simulink model "sf_boiler"  (R2025b)
settings: Solver=ode45  StartTime=0.0  StopTime=1400  RelTol=1e-3  EnableMultiTasking=on
settings Model: ExtModeTrigMode=oneshot  ExtModeArmWhenConnect=off  ExtModeAutoUpdateStatusClock=off  Creator=The MathWorks, Inc.  LastModifiedBy=The MathWorks, Inc.
settings SolverCC: AlgebraicLoopSolver=TrustRegion  InsertRTBMode=Auto
settings DataIOCC: SaveFormat=Array  SaveOutput=off  SaveTime=off  ReturnWorkspaceOutputs=off  SignalLoggingName=sigsOut
settings OptimizationCC: BlockReduction=off  BooleanDataType=off  ReuseModelBlockBuffer=off  ExpressionDepthLimit=2147483647.0  InitFltsAndDblsToZero=on  LifeSpan=1  EfficientTunableParamExpr=on
settings DebuggingCC: SaveWithParameterizedLinksMsg=none  UnderspecifiedInitializationDetection=Classic  MergeDetectMultiDrivingBlocksExec=none  SignalResolutionControl=TryResolveAllWithWarning  MultiTaskDSMMsg=warning  MultiTaskCondExecSysMsg=none  FcnCallInpInsideContextMsg=warning  UnconnectedInputMsg=warning  UnconnectedOutputMsg=warning  UnconnectedLineMsg=warning  StateNameClashWarn=warning  SFUnexpectedBacktrackingDiag=warning  SFNoUnconditionalDefaultTransitionDiag=warning  SFExecutionAtInitializationDiag=none  ArithmeticOperatorsInVariantConditions=warning
settings HardwareCC: ProdBitPerPointer=32.0  ProdBitPerSizeT=32.0  ProdBitPerPtrDiffT=32.0  ProdLargestAtomicFloat=None  ProdIntDivRoundTo=Undefined  ProdEndianess=Unspecified  ProdWordSize=32.0  ProdHWDeviceType=ASIC/FPGA  TargetUnknown=on  ProdEqTarget=off
settings ModelReferenceCC: EnableRefExpFcnMdlSchedulingChecks=on  PropagateSignalLabelsOutOfModel=off
settings SFSimCC: SFSimEcho=off  SimUseLocalCustomCode=off  SimParseCustomCode=off  CustomCodeUndefinedFunction=UseInterfaceOnly
settings RTWCC: SystemTargetFile=ert.tlc  GenCodeOnly=on  TemplateMakefile=ert_default_tmf  GenerateReport=on  RTWVerbose=off  RTWUseLocalCustomCode=off  IncludeHyperlinkInReport=on  LaunchReport=on  GPUComputeCapability=3.5  DLArmComputeVersion=19.05
settings CodeAppCC: IgnoreCustomStorageClasses=off  CustomSymbolStrType=$N$R$M  CustomSymbolStrModelFcn=$N  StateflowObjectComments=on  InternalIdentifier=Classic
settings ERTTargetCC: InlinedParameterPlacement=Hierarchical  ERTCustomFileTemplate=example_file_process.tlc  ConvertIfToSwitch=off  SuppressUnreachableDefaultCases=off  TargetFcnLib=ansi_tfl_tmw.mat  MultiwordLength=2048.0  GenerateSampleERTMain=on  SupportContinuousTime=on  SupportNonInlinedSFcns=on
settings ConfigComp: CovMetricSettings=dcmtr  CovSaveCumulativeToWorkspaceVar=on  CovSaveSingleToWorkspaceVar=on  CovExternalEMLEnable=off  CovSFcnEnable=off

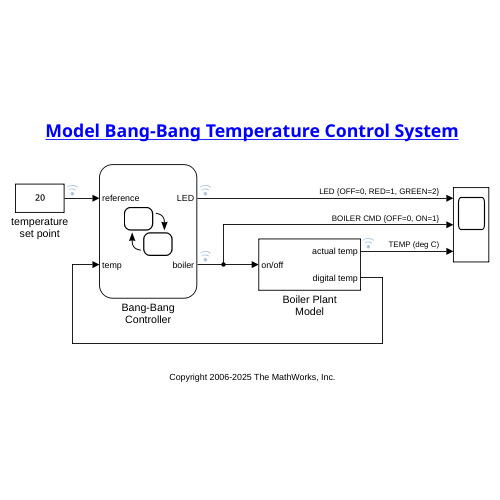
[thumbnail: Simulink's stored preview of the top-level diagram]
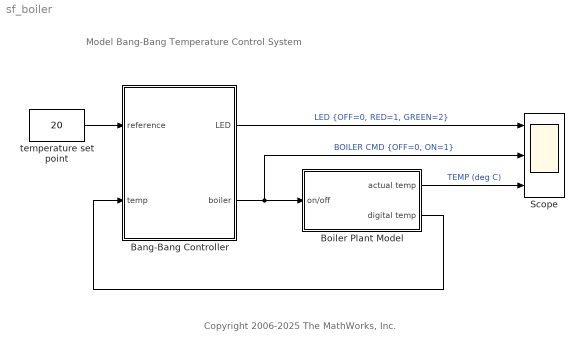
== system sf_boiler ==
  note: Copyright 2006-2025 The MathWorks, Inc.
  note: Model Bang-Bang Temperature Control System
  Bang-Bang Controller : Stateflow chart  TreatAsAtomicUnit=on
  Boiler Plant Model : Subsystem
  Scope : Scope  NumInputPorts=3
      settings: ActiveDisplayYMinimum=0  ActiveDisplayYMaximum=2
  temperature set point : Constant  Value=20  OutDataTypeStr=Inherit: Inherit via back propagation
  wires:
  Bang-Bang Controller/2(" boiler") -> Scope/2, Boiler Plant Model/1(on/off)  "BOILER CMD {OFF=0, ON=1}"
  temperature set point/1 -> Bang-Bang Controller/1(reference)
  Boiler Plant Model/2(digital temp) -> Bang-Bang Controller/2(temp)
  Boiler Plant Model/1(actual temp) -> Scope/3  "TEMP (deg C)"
  Bang-Bang Controller/1(LED) -> Scope/1  "LED {OFF=0, RED=1, GREEN=2}"

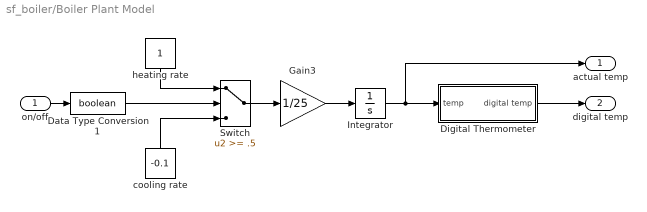
== system sf_boiler/Boiler Plant Model ==
  on/off : Inport
  Data Type Conversion1 : DataTypeConversion  OutDataTypeStr=boolean
  Digital Thermometer : Subsystem
  Gain3 : Gain  Gain=1/25  SaturateOnIntegerOverflow=on  OutDataTypeStr=Inherit: Same as input  ParamDataTypeStr=Inherit: Same as input
  Integrator : Integrator  InitialCondition=15  ZeroCross=off
  Switch : Switch  Threshold=.5
  cooling rate : Constant  Value=-0.1
  heating rate : Constant
  actual temp : Outport  VectorParamsAs1DForOutWhenUnconnected=off
  digital temp : Outport  Port=2  VectorParamsAs1DForOutWhenUnconnected=off
  wires:
  Gain3/1 -> Integrator/1
  cooling rate/1 -> Switch/3
  heating rate/1 -> Switch/1
  Switch/1 -> Gain3/1
  on/off/1 -> Data Type Conversion1/1
  Data Type Conversion1/1 -> Switch/2
  Integrator/1 -> actual temp/1, Digital Thermometer/1(temp)
  Digital Thermometer/1(digital temp) -> digital temp/1

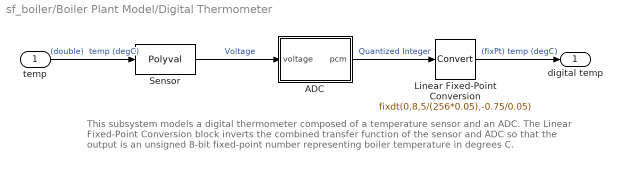
== system sf_boiler/Boiler Plant Model/Digital Thermometer ==
  note: This subsystem models a digital thermometer composed of a temperature sensor and an ADC.
      | The Linear Fixed-Point Conversion block inverts the combined transfer function of the sensor and ADC
      | so that the output is an unsigned 8-bit fixed-point number representing boiler temperature in degrees C.
  temp : Inport
  ADC : Subsystem
      mask Display: fprintf('ADC\n8-bit\n0-5V');
  Linear Fixed-Point Conversion : DataTypeConversion  OutDataTypeStr=fixdt(0,8,5/(256*0.05),-0.75/0.05)  ConvertRealWorld=Stored Integer (SI)  SaturateOnIntegerOverflow=off  RndMeth=Floor
  Sensor : Polyval  Coefs="[ 0.05     0.75 ]"
  digital temp : Outport  VectorParamsAs1DForOutWhenUnconnected=off
  wires:
  temp/1 -> Sensor/1  "(double)  temp (degC)"
  Linear Fixed-Point Conversion/1 -> digital temp/1  "(fixPt) temp (degC)"
  Sensor/1 -> ADC/1(voltage)  "Voltage"
  ADC/1(pcm) -> Linear Fixed-Point Conversion/1  "Quantized Integer"

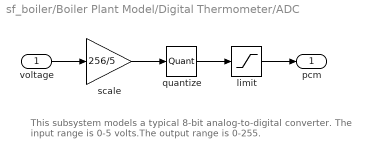
== system sf_boiler/Boiler Plant Model/Digital Thermometer/ADC ==
  note: This subsystem models a typical 8-bit analog-to-digital converter. The input range is 0-5 volts.The output range is 0-255.
  voltage : Inport
  limit : Saturate  UpperLimit=255  LowerLimit=0
  quantize : Quantizer  QuantizationInterval=1
  scale : Gain  Gain=256/5  SaturateOnIntegerOverflow=on  OutDataTypeStr=Inherit: Same as input  ParamDataTypeStr=Inherit: Same as input
  pcm : Outport  VectorParamsAs1DForOutWhenUnconnected=off
  wires:
  voltage/1 -> scale/1
  quantize/1 -> limit/1
  scale/1 -> quantize/1
  limit/1 -> pcm/1

== stateflow chart sf_boiler/Bang-Bang Controller ==
  settings: updateMethod=DISCRETE  sampleTime=1
  state Heater [group]
    state Off
      en: LED = RED;
      state Flash
        en: flash_LED()
      Flash -> Flash : after(5,sec)
    state On
      en,du: flash_LED()
      (history)
      state HIGH
      state NORM
      (default) -> HIGH
      NORM -> 74 : [warm()]
      HIGH -> NORM : [warm()]
    (default) -> Off
    On -> Off : after(20,sec)
    Off -> On : after(40,sec)[cold()]
    75 -> Off
  state flash_LED [function]
    (default) -> (junction 60)
    (junction 60) -> (junction 62) [order 1] : [boiler == ON]
    (junction 60) -> (junction 66) [order 2] : {color=RED}
    (junction 62) -> (junction 64) : {color=GREEN}
    (junction 64) -> (junction 66)
    (junction 66) -> (junction 37)
    (junction 37) -> (junction 38) [order 1] : [LED == color]
    (junction 37) -> (junction 31) [order 2] : {LED=color}
    (junction 38) -> (junction 42) : {LED=OFF}
  state b = cold [function]
    (default) -> (junction 39) : { b = temp<=reference}
  state b = warm [function]
    (default) -> (junction 72) : {b = ~cold()}
  data: b function_output boolean; b function_output boolean; LED output int8; color local int8; reference input fixdt(0,8,1,-15); GREEN constant int8 =2; OFF constant int8 =0; ON constant int8 =1; RED constant int8 =1; temp input fixdt(0,8,5/(256*0.05),-0.75/0.05); boiler output boolean
